simulink model "si_mimo_mpc"  (R2025b)
settings: Solver=FixedStepDiscrete  StartTime=0.0  StopTime=20  FixedStep=.2  RelTol=1e-3
settings Model: Creator=runner  LastModifiedBy=runner

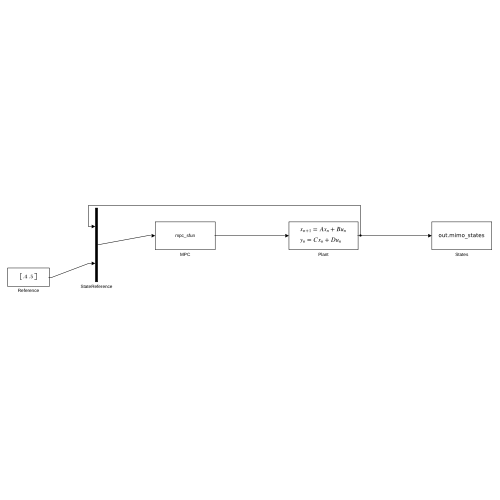
[thumbnail: Simulink's stored preview of the top-level diagram]
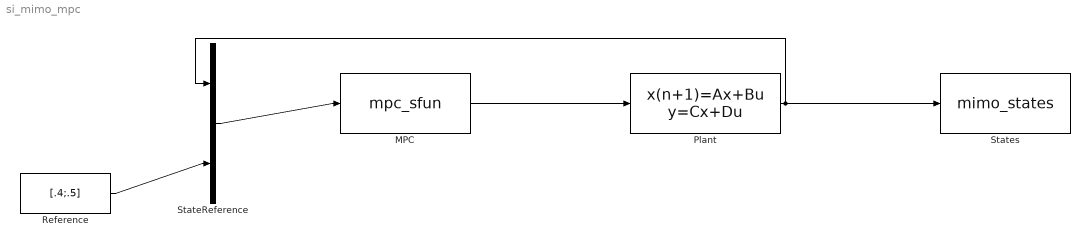
== system si_mimo_mpc ==
  MPC : S-Function  FunctionName=mpc_sfun  SFunctionDeploymentMode=off  EnableBusSupport=off
  Plant : DiscreteStateSpace  A=diag([.96 .94])  B=[.04 .012;.01 .05]  C=eye(2)  D=zeros(2)  SampleTime=.2
  Reference : Constant  Value=[.4;.5]
  StateReference : Mux  Inputs=2
  States : ToWorkspace  VariableName=mimo_states  SaveFormat=Structure With Time  SampleTime=-1
  wires:
  Reference/1 -> StateReference/2
  StateReference/1 -> MPC/1
  MPC/1 -> Plant/1
  Plant/1 -> States/1, StateReference/1
